simulink model "finalmodel1"  (R2024b)
settings: Solver=FixedStepDiscrete  StartTime=0.0  StopTime=110  FixedStep=SampleTime  MaxStep=1e-3  RelTol=1e-4  AbsTol=1e-3
InitFcn:
  | Ts=50e-6; SampleTime=50e-6; PSSMODEL=1;
  | MB=[1   0.2 30   1.25 40    12 160];
  | 
  | k=[8.3222    2.6014   19.0811    1.9818    3.6841   19.1783  240.6785    2.5684    4.3666   58.7391 7.6960   47.7975    8.7139  296.2463    2.7543    6.5051   47.7755    0.4780   35.4950   18.1866 94.2186]
  | k1=k(1);
  | k2=k(2);
  | k3=k(3);
  | k4=k(4);
  | k5=k(5);
  | k6=k(6);
  | k7=k(7);
  | k8=k(8);
  | k9=k(9);
  | k10=k(10);
  | k11=k(11);
  | k12=k(12);
  | k13=k(13);
  | k14=k(14);
  | k15=k(15);
  | k16=k(16);
  | k17=k(17);
  | k18=k(18);
  | k19=k(19);
  | k20=k(20);
  | k21=k(21);
undefined symbols (not defined in the file or in its folder): dEgdT, DiscIntNeverNeededParam, EgRef, gcbh, Rsh_array5pc, sigbuilder_block, sps_rtmsupport, Tref_K, VT_ref
libraries: spsThreePhaseVIMeasurementLib x14, spsLoadFlowBusLib x9, spsThreePhasePISectionLineLib x6, spsSeriesRLCBranchLib x5, spsThreePhaseTransformerTwoWindingsLib x4, slpidlib x4, spsThreePhaseParallelRLCLoadLib x4, spsThreePhaseSeriesRLCBranchLib x3, spsAlphaBetaZerotodq0Lib x2, spsSynchronousMachinepuStandardLib x2, spsExcitationSystemLib x2, spsMultiBandPowerSystemStabilizerLib x2
(part 9 of 9)

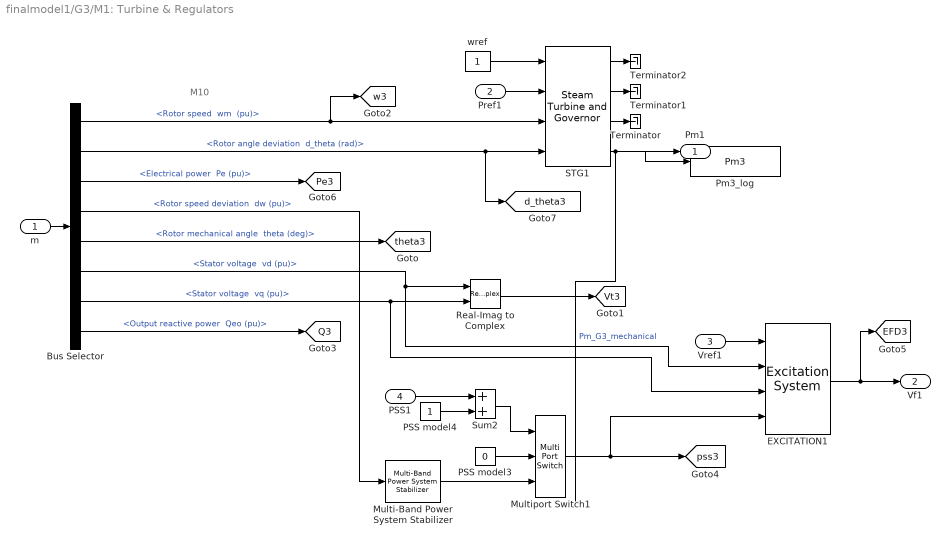
== system finalmodel1/G3/M1: Turbine & Regulators ==
  note: M10
  m : Inport  SampleTime=SampleTime
  Pref1 : Inport  Port=2  SampleTime=SampleTime
  Vref1 : Inport  Port=3  SampleTime=SampleTime
  PSS1 : Inport  Port=4  SampleTime=SampleTime
  Bus Selector : BusSelector  OutputSignals="Mechanical.Rotor speed  wm  (pu),Mechanical.Rotor angle deviation  d_theta (rad),Mechanical.Electrical power  Pe (pu),Mechanical.Rotor speed deviation  dw (pu),Mechanical.Rotor mechanical angle  theta (deg),dq0 components.Stator voltage  vd (pu),dq0 components.Stator voltage  vq (pu),Output reactive power  Qeo (pu)"
  EXCITATION1 : spsExcitationSystemLib/Excitation System  tr=0.01  reg=[20 .2]  exc=[ 1, 0.314 ]  tgr=[ 10 1]  damp=[ 0.063, 0.35 ]  sat=[ 0, 0 ]  lim="[ -5 5  0 ]"  v0=[1.025 1.2647]
      link override Model: Ts=SampleTime
      link override Model/Damping kfd.s // (tfd.s +1)/1st-Order Discrete Filter: Ts=SampleTime
      link override Model/Damping kfd.s // (tfd.s +1)/1st-Order Discrete Filter/Discrete State-Space: SampleTime=SampleTime
      link override Model/Exciter  1 // (te.s + ke)/1st order Lowpass: Ts=SampleTime
      link override Model/Exciter  1 // (te.s + ke)/1st order Lowpass/Discrete State-Space: SampleTime=SampleTime
      link override Model/Lead Lag Compensator tc.s+1 // tb.s+1: Ts=SampleTime
      link override Model/Lead Lag Compensator tc.s+1 // tb.s+1/Discrete State-Space: SampleTime=SampleTime
      link override Model/Low Pass Filter 1 // (tr.s +1) (with IC): Ts=SampleTime
      link override Model/Low Pass Filter 1 // (tr.s +1) (with IC)/Discrete State-Space: SampleTime=SampleTime
      link override Model/Main Regulator ka // (ta.s +1)/1st order Lowpass: Ts=SampleTime
      link override Model/Main Regulator ka // (ta.s +1)/1st order Lowpass/Discrete State-Space: SampleTime=SampleTime
      link override Model/Positive Sequence Voltage: Expr=sqrt(abs(u(1)^2 + u(2)^2))
      link override Model/Unit Delay1: SampleTime=SampleTime
      link override Model/Unit Delay2: SampleTime=SampleTime
      settings: LibrarySourceBlock=sps_lib/Electrical Machines/Synchronous Machine Control/Excitation System
  Multi-Band Power System Stabilizer : spsMultiBandPowerSystemStabilizerLib/Multi-Band Power System Stabilizer  OperationMode=Simplified settings  Kg=k1  GL=[k2 k3]  GI=[k4 k5]  GH=[k6 k7]  GLd=[66 66 9.4]  TcLF=[1.667 2 0 0 0 0 2 2.4 0 0 0 0 1 1]  GId=[66 66 47.6]  TcIF=[1 1 0.25 0.3 0 0 1 1 0.3 0.36 0 0 0 0]  GHd=[66 66 233]  TcHF="[0.01 0.012 0 0 0 0  0.012 0.0144 0 0 0 0 1 1]"  LIM=[.075 .15 .15 .15]  Plot_On=off  MagdB_On=off  FreqRange=logspace(-2,2,500)
      link override Model/Discrete Lead-Lag1: Ts=SampleTime
      link override Model/Discrete Lead-Lag1/Discrete State-Space: SampleTime=SampleTime
      link override Model/Discrete Lead-Lag2: Ts=SampleTime
      link override Model/Discrete Lead-Lag2/Discrete State-Space: SampleTime=SampleTime
      link override Model/Discrete Lead-Lag3: Ts=SampleTime
      link override Model/Discrete Lead-Lag3/Discrete State-Space: SampleTime=SampleTime
      link override Model/Discrete Lead-Lag4: Ts=SampleTime
      link override Model/Discrete Lead-Lag4/Discrete State-Space: SampleTime=SampleTime
      link override Model/Discrete Lead-Lag5: Ts=SampleTime
      link override Model/Discrete Lead-Lag5/Discrete State-Space: SampleTime=SampleTime
      link override Model/Discrete Lead-Lag6: Ts=SampleTime
      link override Model/Discrete Lead-Lag6/Discrete State-Space: SampleTime=SampleTime
      link override Model/HF speed sensor: Ts=SampleTime
      link override Model/HF speed sensor/Discrete State-Space: SampleTime=SampleTime
      link override Model/LF and IF speed sensor: Ts=SampleTime
      link override Model/LF and IF speed sensor/Discrete State-Space: SampleTime=SampleTime
      link override Model/Transfer function for detailed model (HF)/Transfer functions for detailed stabilizer/Discrete Lead-Lag1: Ts=SampleTime
      link override Model/Transfer function for detailed model (HF)/Transfer functions for detailed stabilizer/Discrete Lead-Lag1/Discrete State-Space: SampleTime=SampleTime
      link override Model/Transfer function for detailed model (HF)/Transfer functions for detailed stabilizer/Discrete Lead-Lag2: Ts=SampleTime
      link override Model/Transfer function for detailed model (HF)/Transfer functions for detailed stabilizer/Discrete Lead-Lag2/Discrete State-Space: SampleTime=SampleTime
      link override Model/Transfer function for detailed model (HF)/Transfer functions for detailed stabilizer1/Discrete Lead-Lag1: Ts=SampleTime
      link override Model/Transfer function for detailed model (HF)/Transfer functions for detailed stabilizer1/Discrete Lead-Lag1/Discrete State-Space: SampleTime=SampleTime
      link override Model/Transfer function for detailed model (HF)/Transfer functions for detailed stabilizer1/Discrete Lead-Lag2: Ts=SampleTime
      link override Model/Transfer function for detailed model (HF)/Transfer functions for detailed stabilizer1/Discrete Lead-Lag2/Discrete State-Space: SampleTime=SampleTime
      link override Model/Transfer function for detailed model (IF)/Transfer functions for detailed stabilizer/Discrete Lead-Lag1: Ts=SampleTime
      link override Model/Transfer function for detailed model (IF)/Transfer functions for detailed stabilizer/Discrete Lead-Lag1/Discrete State-Space: SampleTime=SampleTime
      link override Model/Transfer function for detailed model (IF)/Transfer functions for detailed stabilizer/Discrete Lead-Lag2: Ts=SampleTime
      link override Model/Transfer function for detailed model (IF)/Transfer functions for detailed stabilizer/Discrete Lead-Lag2/Discrete State-Space: SampleTime=SampleTime
      link override Model/Transfer function for detailed model (IF)/Transfer functions for detailed stabilizer1/Discrete Lead-Lag1: Ts=SampleTime
      link override Model/Transfer function for detailed model (IF)/Transfer functions for detailed stabilizer1/Discrete Lead-Lag1/Discrete State-Space: SampleTime=SampleTime
      link override Model/Transfer function for detailed model (IF)/Transfer functions for detailed stabilizer1/Discrete Lead-Lag2: Ts=SampleTime
      link override Model/Transfer function for detailed model (IF)/Transfer functions for detailed stabilizer1/Discrete Lead-Lag2/Discrete State-Space: SampleTime=SampleTime
      link override Model/Transfer function for detailed model (LF)/Transfer functions for detailed stabilizer/Discrete Lead-Lag1: Ts=SampleTime
      link override Model/Transfer function for detailed model (LF)/Transfer functions for detailed stabilizer/Discrete Lead-Lag1/Discrete State-Space: SampleTime=SampleTime
      link override Model/Transfer function for detailed model (LF)/Transfer functions for detailed stabilizer/Discrete Lead-Lag2: Ts=SampleTime
      link override Model/Transfer function for detailed model (LF)/Transfer functions for detailed stabilizer/Discrete Lead-Lag2/Discrete State-Space: SampleTime=SampleTime
      link override Model/Transfer function for detailed model (LF)/Transfer functions for detailed stabilizer1/Discrete Lead-Lag1: Ts=SampleTime
      link override Model/Transfer function for detailed model (LF)/Transfer functions for detailed stabilizer1/Discrete Lead-Lag1/Discrete State-Space: SampleTime=SampleTime
      link override Model/Transfer function for detailed model (LF)/Transfer functions for detailed stabilizer1/Discrete Lead-Lag2: Ts=SampleTime
      link override Model/Transfer function for detailed model (LF)/Transfer functions for detailed stabilizer1/Discrete Lead-Lag2/Discrete State-Space: SampleTime=SampleTime
      settings: LibrarySourceBlock=|
      | sps_lib/Electrical Machines/Synchronous Machine Control/Multi-Band
      | Power System Stabilizer
  Multiport Switch1 : MultiPortSwitch  Inputs=2  SampleTime=SampleTime  SaturateOnIntegerOverflow=off
  PSS model3 : Constant  Value=0  SampleTime=SampleTime
  PSS model4 : Constant  SampleTime=SampleTime
  Pm3_log : ToWorkspace  VariableName=Pm3  SaveFormat=Timeseries  SampleTime=-1
  Real-Imag to Complex : RealImagToComplex  SampleTime=SampleTime
  STG1 : spsSteamTurbineandGovernorLib/Steam Turbine and Governor  gentype=Tandem-compound (single mass)  reg1="[ 1  0.05    0 ]"  reg2="[ 0.001  0.15 ]"  reg3="[ -0.1  0.1  0  4.496 ]"  N=3600  turb1="[ 0  10   3.3   0.5   ]"  turb2="[   0   0.36    0.36   0.28   ]"  HA="[ 0.046  1.430  1.465   0.192 ]"  KA="[ 90.44  53.88  64.59   62.94  ]"  DA="[ 0.0115  0.3575  0.3663   0.0137  ]"  ini1=0.66512  ini2=[0.779316,-31.4247]
      link override Model/4 mass shaft/1 mass/Mass2: Ts=SampleTime
      link override Model/4 mass shaft/1 mass/Mass2/Ad*x(k-1): SampleTime=SampleTime
      link override Model/4 mass shaft/1 mass/Mass2/Bd*(u(k)+ u(k-1)): SampleTime=SampleTime
      link override Model/4 mass shaft/1 mass/Mass2/Delay_u: SampleTime=SampleTime
      link override Model/4 mass shaft/1 mass/Mass2/Delay_x: SampleTime=SampleTime
      link override Model/4 mass shaft/1 mass/Mass2/Digital Clock: SampleTime=SampleTime
      link override Model/4 mass shaft/1 mass/Mass2/Prediction/Unit Delay3: SampleTime=SampleTime
      link override Model/4 mass shaft/2 masses/Mass2: Ts=SampleTime
      link override Model/4 mass shaft/2 masses/Mass2/Ad*x(k-1): SampleTime=SampleTime
      link override Model/4 mass shaft/2 masses/Mass2/Bd*(u(k)+ u(k-1)): SampleTime=SampleTime
      link override Model/4 mass shaft/2 masses/Mass2/Delay_u: SampleTime=SampleTime
      link override Model/4 mass shaft/2 masses/Mass2/Delay_x: SampleTime=SampleTime
      link override Model/4 mass shaft/2 masses/Mass2/Digital Clock: SampleTime=SampleTime
      link override Model/4 mass shaft/2 masses/Mass2/Prediction/Unit Delay3: SampleTime=SampleTime
      link override Model/4 mass shaft/2 masses/Mass3: Ts=SampleTime
      link override Model/4 mass shaft/2 masses/Mass3/Ad*x(k-1): SampleTime=SampleTime
      link override Model/4 mass shaft/2 masses/Mass3/Bd*(u(k)+ u(k-1)): SampleTime=SampleTime
      link override Model/4 mass shaft/2 masses/Mass3/Delay_u: SampleTime=SampleTime
      link override Model/4 mass shaft/2 masses/Mass3/Delay_x: SampleTime=SampleTime
      link override Model/4 mass shaft/2 masses/Mass3/Digital Clock: SampleTime=SampleTime
      link override Model/4 mass shaft/2 masses/Mass3/Prediction/Unit Delay3: SampleTime=SampleTime
      link override Model/4 mass shaft/3 masses/Mass2: Ts=SampleTime
      link override Model/4 mass shaft/3 masses/Mass2/Ad*x(k-1): SampleTime=SampleTime
      link override Model/4 mass shaft/3 masses/Mass2/Bd*(u(k)+ u(k-1)): SampleTime=SampleTime
      link override Model/4 mass shaft/3 masses/Mass2/Delay_u: SampleTime=SampleTime
      link override Model/4 mass shaft/3 masses/Mass2/Delay_x: SampleTime=SampleTime
      link override Model/4 mass shaft/3 masses/Mass2/Digital Clock: SampleTime=SampleTime
      link override Model/4 mass shaft/3 masses/Mass2/Prediction/Unit Delay3: SampleTime=SampleTime
      link override Model/4 mass shaft/3 masses/Mass3: Ts=SampleTime
      link override Model/4 mass shaft/3 masses/Mass3/Ad*x(k-1): SampleTime=SampleTime
      link override Model/4 mass shaft/3 masses/Mass3/Bd*(u(k)+ u(k-1)): SampleTime=SampleTime
      link override Model/4 mass shaft/3 masses/Mass3/Delay_u: SampleTime=SampleTime
      link override Model/4 mass shaft/3 masses/Mass3/Delay_x: SampleTime=SampleTime
      link override Model/4 mass shaft/3 masses/Mass3/Digital Clock: SampleTime=SampleTime
      link override Model/4 mass shaft/3 masses/Mass3/Prediction/Unit Delay3: SampleTime=SampleTime
      link override Model/4 mass shaft/3 masses/Mass4: Ts=SampleTime
      link override Model/4 mass shaft/3 masses/Mass4/Ad*x(k-1): SampleTime=SampleTime
      link override Model/4 mass shaft/3 masses/Mass4/Bd*(u(k)+ u(k-1)): SampleTime=SampleTime
      link override Model/4 mass shaft/3 masses/Mass4/Delay_u: SampleTime=SampleTime
      link override Model/4 mass shaft/3 masses/Mass4/Delay_x: SampleTime=SampleTime
      link override Model/4 mass shaft/3 masses/Mass4/Digital Clock: SampleTime=SampleTime
      link override Model/4 mass shaft/3 masses/Mass4/Prediction/Unit Delay3: SampleTime=SampleTime
      link override Model/4 mass shaft/4 masses/Mass2: Ts=SampleTime
      link override Model/4 mass shaft/4 masses/Mass2/Ad*x(k-1): SampleTime=SampleTime
      link override Model/4 mass shaft/4 masses/Mass2/Bd*(u(k)+ u(k-1)): SampleTime=SampleTime
      link override Model/4 mass shaft/4 masses/Mass2/Delay_u: SampleTime=SampleTime
      link override Model/4 mass shaft/4 masses/Mass2/Delay_x: SampleTime=SampleTime
      link override Model/4 mass shaft/4 masses/Mass2/Digital Clock: SampleTime=SampleTime
      link override Model/4 mass shaft/4 masses/Mass2/Prediction/Unit Delay3: SampleTime=SampleTime
      link override Model/4 mass shaft/4 masses/Mass3: Ts=SampleTime
      link override Model/4 mass shaft/4 masses/Mass3/Ad*x(k-1): SampleTime=SampleTime
      link override Model/4 mass shaft/4 masses/Mass3/Bd*(u(k)+ u(k-1)): SampleTime=SampleTime
      link override Model/4 mass shaft/4 masses/Mass3/Delay_u: SampleTime=SampleTime
      link override Model/4 mass shaft/4 masses/Mass3/Delay_x: SampleTime=SampleTime
      link override Model/4 mass shaft/4 masses/Mass3/Digital Clock: SampleTime=SampleTime
      link override Model/4 mass shaft/4 masses/Mass3/Prediction/Unit Delay3: SampleTime=SampleTime
      link override Model/4 mass shaft/4 masses/Mass4: Ts=SampleTime
      link override Model/4 mass shaft/4 masses/Mass4/Ad*x(k-1): SampleTime=SampleTime
      link override Model/4 mass shaft/4 masses/Mass4/Bd*(u(k)+ u(k-1)): SampleTime=SampleTime
      link override Model/4 mass shaft/4 masses/Mass4/Delay_u: SampleTime=SampleTime
      link override Model/4 mass shaft/4 masses/Mass4/Delay_x: SampleTime=SampleTime
      link override Model/4 mass shaft/4 masses/Mass4/Digital Clock: SampleTime=SampleTime
      link override Model/4 mass shaft/4 masses/Mass4/Prediction/Unit Delay3: SampleTime=SampleTime
      link override Model/4 mass shaft/4 masses/Mass5: Ts=SampleTime
      link override Model/4 mass shaft/4 masses/Mass5/Ad*x(k-1): SampleTime=SampleTime
      link override Model/4 mass shaft/4 masses/Mass5/Bd*(u(k)+ u(k-1)): SampleTime=SampleTime
      link override Model/4 mass shaft/4 masses/Mass5/Delay_u: SampleTime=SampleTime
      link override Model/4 mass shaft/4 masses/Mass5/Delay_x: SampleTime=SampleTime
      link override Model/4 mass shaft/4 masses/Mass5/Digital Clock: SampleTime=SampleTime
      link override Model/4 mass shaft/4 masses/Mass5/Prediction/Unit Delay3: SampleTime=SampleTime
      link override Model/speed regulator/Servo-motor Position: SampleTime=SampleTime
      link override Model/speed regulator/Speed Relay: Ts=SampleTime
      link override Model/speed regulator/Speed Relay/In: SampleTime=SampleTime
      link override Model/speed regulator/Speed Relay/Model/Delay_x: SampleTime=SampleTime
      link override Model/speed regulator/Speed Relay/Out: SampleTime=SampleTime
      link override Model/steam turbine/Stage 1/Constant4: SampleTime=SampleTime
      link override Model/steam turbine/Stage 1/Stage1/Stage1: Ts=SampleTime
      link override Model/steam turbine/Stage 1/Stage1/Stage1/In: SampleTime=SampleTime
      link override Model/steam turbine/Stage 1/Stage1/Stage1/Model/Delay_x: SampleTime=SampleTime
      link override Model/steam turbine/Stage 1/Stage1/Stage1/Out: SampleTime=SampleTime
      link override Model/steam turbine/Stage 2 /Constant3: SampleTime=SampleTime
      link override Model/steam turbine/Stage 2 /Stage2/Stage2: Ts=SampleTime
      link override Model/steam turbine/Stage 2 /Stage2/Stage2/In: SampleTime=SampleTime
      link override Model/steam turbine/Stage 2 /Stage2/Stage2/Model/Delay_x: SampleTime=SampleTime
      link override Model/steam turbine/Stage 2 /Stage2/Stage2/Out: SampleTime=SampleTime
      link override Model/steam turbine/Stage 3/Constant2: SampleTime=SampleTime
      link override Model/steam turbine/Stage 3/Stage3/Stage3: Ts=SampleTime
      link override Model/steam turbine/Stage 3/Stage3/Stage3/In: SampleTime=SampleTime
      link override Model/steam turbine/Stage 3/Stage3/Stage3/Model/Delay_x: SampleTime=SampleTime
      link override Model/steam turbine/Stage 3/Stage3/Stage3/Out: SampleTime=SampleTime
      link override Model/steam turbine/Stage 4/Constant1: SampleTime=SampleTime
      link override Model/steam turbine/Stage 4/Stage4/Stage4: Ts=SampleTime
      link override Model/steam turbine/Stage 4/Stage4/Stage4/In: SampleTime=SampleTime
      link override Model/steam turbine/Stage 4/Stage4/Stage4/Model/Delay_x: SampleTime=SampleTime
      link override Model/steam turbine/Stage 4/Stage4/Stage4/Out: SampleTime=SampleTime
      settings: LibrarySourceBlock=|
      | sps_lib/Electrical Machines/Synchronous Machine Control/Steam Turbine
      | and Governor
  Sum2 : Sum  InputSameDT=on  SaturateOnIntegerOverflow=on  SampleTime=SampleTime  OutDataTypeStr=Inherit: Same as first input
  Terminator : Terminator
  Terminator1 : Terminator
  Terminator2 : Terminator
  wref : Constant  SampleTime=SampleTime
  Pm1 : Outport  SampleTime=SampleTime  InitialOutput=0
  Vf1 : Outport  Port=2  SampleTime=SampleTime  InitialOutput=0
  tag scope: EFD3=global, Pe3=global, Q3=global, Vt3=global, d_theta3=global, pss3=global, theta3=global, w3=global
  wires:
  Bus Selector/4 -> Multi-Band Power System Stabilizer/1  "<Rotor speed deviation  dw (pu)>"
  Multiport Switch1/1 -> EXCITATION1/4, [pss3]
  PSS model3/1 -> Multiport Switch1/2
  Multi-Band Power System Stabilizer/1 -> Multiport Switch1/3
  PSS model4/1 -> Sum2/2
  Sum2/1 -> Multiport Switch1/1
  PSS1/1 -> Sum2/1
  Bus Selector/8 -> [Q3]  "<Output reactive power  Qeo (pu)>"
  Bus Selector/3 -> [Pe3]  "<Electrical power  Pe (pu)>"
  Bus Selector/2 -> STG1/4, [d_theta3]  "<Rotor angle deviation  d_theta (rad)>"
  Bus Selector/1 -> STG1/3, [w3]  "<Rotor speed  wm  (pu)>"
  STG1/1 -> Terminator2/1
  STG1/2 -> Terminator1/1
  STG1/3 -> Terminator/1
  Bus Selector/6 -> EXCITATION1/2, Real-Imag to Complex/1  "<Stator voltage  vd (pu)>"
  Bus Selector/5 -> [theta3]  "<Rotor mechanical angle  theta (deg)>"
  Real-Imag to Complex/1 -> [Vt3]
  EXCITATION1/1 -> [EFD3], Vf1/1
  Vref1/1 -> EXCITATION1/1
  m/1 -> Bus Selector/1
  Pref1/1 -> STG1/2
  wref/1 -> STG1/1
  Bus Selector/7 -> Real-Imag to Complex/2, EXCITATION1/3  "<Stator voltage  vq (pu)>"
  STG1/4 -> Pm1/1, Pm3_log/1  "Pm_G3_mechanical"

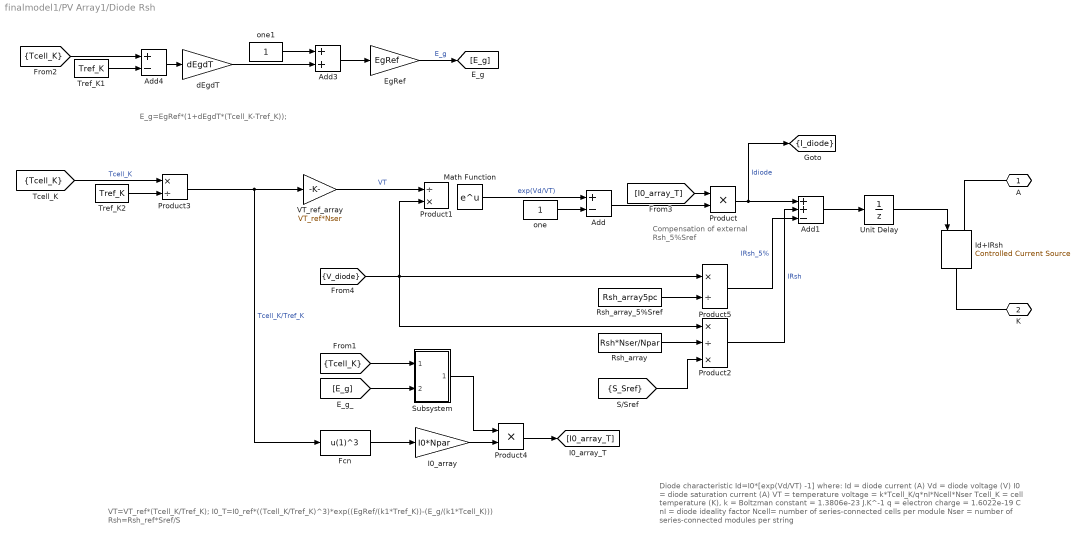
== system finalmodel1/PV Array1/Diode Rsh ==
  note: E_g=EgRef*(1+dEgdT*(Tcell_K-Tref_K));
  note: VT=VT_ref*(Tcell_K/Tref_K);
      | I0_T=I0_ref*((Tcell_K/Tref_K)^3)*exp((EgRef/(k1*Tref_K))-(E_g/(k1*Tcell_K)))
      | Rsh=Rsh_ref*Sref/S
  note: Diode characteristic
      |    Id=I0*[exp(Vd/VT) -1]
      |
      | where:
      |      Id = diode current (A)
      |      Vd = diode voltage (V)
      |      I0 = diode saturation current (A)
      |      VT = temperature voltage = k*Tcell_K/q*nI*Ncell*Nser
      | Tcell_K = cell temperature (K),
      |       k = Boltzman constant = 1.3806e-23 J.K^-1
      |       q = electron charge = 1.6022e-19 C
      |      nI = diode ideality factor
      |    Ncell= number of series-connected cells per module
      |    Nser = number of series-connected modules per string
  note: Compensation of
      | external Rsh_5%Sref
  Add : Sum  Inputs=+-
  Add1 : Sum  Inputs=++-
  Add3 : Sum
  Add4 : Sum  Inputs=+-
  EgRef : Gain  Gain=EgRef
  Fcn : Fcn  Expr=u(1)^3
  I0_array : Gain  Gain=I0*Npar
  Id+IRsh : spsControlledCurrentSourceLib/Controlled Current Source  Initialize=on  Source_Type=AC  Amplitude=0  Phase=0  Frequency=0  Measurements=None
  Math Function : Math  SignedPower=on  OutputSignalType=real
  Product : Product  RndMeth=Zero
  Product1 : Product  Inputs=/*  RndMeth=Zero
  Product2 : Product  Inputs=*/*  RndMeth=Zero
  Product3 : Product  Inputs=*/  RndMeth=Zero
  Product4 : Product  Inputs=**  RndMeth=Zero
  Product5 : Product  Inputs=*/  RndMeth=Zero
  Rsh_array : Constant  Value=Rsh*Nser/Npar
  Rsh_array_5%Sref : Constant  Value=Rsh_array5pc
  Subsystem : Subsystem
  Tref_K1 : Constant  Value=Tref_K
  Tref_K2 : Constant  Value=Tref_K
  Unit Delay : UnitDelay  SampleTime=SampleTime  HasFrameUpgradeWarning=on
  VT_ref_array : Gain  Gain=VT_ref*Nser
  dEgdT : Gain  Gain=dEgdT
  one : Constant
  one1 : Constant
  A : PMIOPort  Side=Left
  K : PMIOPort  Port=2  Side=Right
  tag scope: I_diode=scoped
  wires:
  [V_diode] -> Product2/1, Product5/1, Product1/2
  [S_Sref] -> Product2/3
  [I0_array_T] -> Product/1
  VT_ref_array/1 -> Product1/1  "VT"
  Add/1 -> Product/2
  Product4/1 -> [I0_array_T]
  Tref_K2/1 -> Product3/2
  [E_g] -> Subsystem/2(E_g)
  [Tcell_K] -> Subsystem/1(Tcell_K)
  Subsystem/1(exp) -> Product4/1
  Tref_K1/1 -> Add4/2
  [Tcell_K] -> Add4/1
  Fcn/1 -> I0_array/1
  I0_array/1 -> Product4/2
  EgRef/1 -> [E_g]  "E_g"
  Add3/1 -> EgRef/1
  dEgdT/1 -> Add3/2
  Add4/1 -> dEgdT/1
  one1/1 -> Add3/1
  Product3/1 -> Fcn/1, VT_ref_array/1  "Tcell_K/Tref_K"
  [Tcell_K] -> Product3/1  "Tcell_K"
  Rsh_array/1 -> Product2/2
  one/1 -> Add/2
  Product/1 -> [I_diode], Add1/1  "Idiode"
  Product2/1 -> Add1/2  "IRsh"
  Math Function/1 -> Add/1  "exp(Vd/VT)"
  Rsh_array_5%Sref/1 -> Product5/2
  Product5/1 -> Add1/3  "IRsh_5%"
  Add1/1 -> Unit Delay/1
  Unit Delay/1 -> Id+IRsh/1
  connections:
  A/RConn1 -- Id+IRsh/LConn1
  Id+IRsh/RConn1 -- K/RConn1

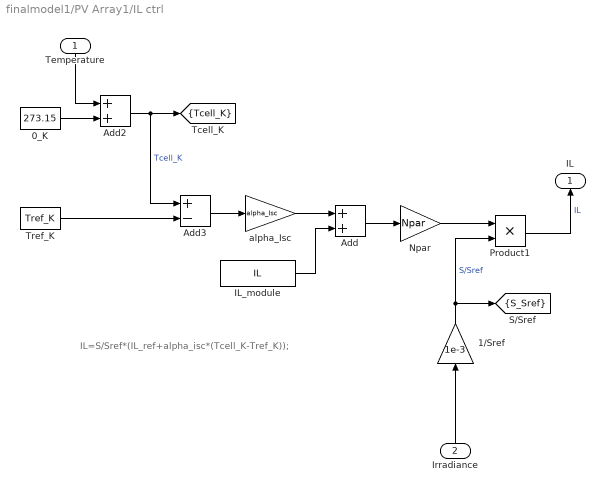
== system finalmodel1/PV Array1/IL ctrl ==
  note: IL=S/Sref*(IL_ref+alpha_isc*(Tcell_K-Tref_K));
  Temperature : Inport
  Irradiance : Inport  Port=2
  0_K : Constant  Value=273.15
  1/Sref : Gain  Gain=1e-3
  Add : Sum
  Add2 : Sum
  Add3 : Sum  Inputs=+-
  IL_module : Constant  Value=IL
  Npar : Gain  Gain=Npar
  Product1 : Product  Inputs=**  RndMeth=Zero
  Tref_K : Constant  Value=Tref_K
  alpha_Isc : Gain  Gain=alpha_Isc
  IL : Outport  VectorParamsAs1DForOutWhenUnconnected=off
  tag scope: S_Sref=scoped, Tcell_K=scoped
  wires:
  1/Sref/1 -> [S_Sref], Product1/2  "S/Sref"
  Npar/1 -> Product1/1
  Add2/1 -> [Tcell_K], Add3/1  "Tcell_K"
  Add/1 -> Npar/1
  0_K/1 -> Add2/2
  IL_module/1 -> Add/2
  Product1/1 -> IL/1  "IL"
  Tref_K/1 -> Add3/2
  Add3/1 -> alpha_Isc/1
  alpha_Isc/1 -> Add/1
  Irradiance/1 -> 1/Sref/1
  Temperature/1 -> Add2/1

== system finalmodel1/PV Array1/Vdiode ==
  note: Vd=V_PV + Rs*I_PV
  I_PV : Inport
  V_PV : Inport  Port=2
  Add1 : Sum
  Product2 : Product  Inputs=**  RndMeth=Zero
  Rs_array_ : Constant  Value=Rs*Nser/Npar
  Vd : Outport  VectorParamsAs1DForOutWhenUnconnected=off
  wires:
  Add1/1 -> Vd/1  "Vd"
  I_PV/1 -> Product2/1
  Product2/1 -> Add1/2
  V_PV/1 -> Add1/1
  Rs_array_/1 -> Product2/2

== system finalmodel1/PV Array1/Diode Rsh/Subsystem ==
  note: exp((EgRef/(k1*Tref_K))-(E_g/(k1*Tcell_K)))
  Tcell_K : Inport
  E_g : Inport  Port=2
  Add : Sum  Inputs=+-
  EgRef : Constant  Value=EgRef/(k1*Tref_K)
  Math Function : Math  SignedPower=on  OutputSignalType=real
  Product : Product  Inputs=*/
  k1 : Gain  Gain=k1
  exp : Outport  VectorParamsAs1DForOutWhenUnconnected=off
  wires:
  Math Function/1 -> exp/1
  Product/1 -> Add/2
  k1/1 -> Product/2
  Tcell_K/1 -> k1/1
  E_g/1 -> Product/1
  EgRef/1 -> Add/1

== matlab function finalmodel1/P&O ==
  settings: updateMethod=DISCRETE  sampleTime=1e-4
  data: Vpv input; D output; Ipv input
function D = PO(Vpv,Ipv)
 Dmax=0.9;
 Dmin=0.1;
 Dinit=0.9;
 deltaD=1e-3;
 persistent Dpre Ppre Vpre;
 
 %first run
     if isempty(Dpre)
         Dpre=Dinit;
         Vpre=0;
         Ppre=0;
     end
 Ppv=Vpv*Ipv;
 dp=Ppv-Ppre;
 dv=Vpv-Vpre;
 
     if dp~=0 
             if(dp>0)
                     if(dv<0)
                         D=Dpre+deltaD;
                     else
                         D=Dpre-deltaD;
                     end     
             else                   
                     if(dv<0)
                         D=Dpre-deltaD;
                     else
                         D=Dpre+deltaD;
                     end
             end   
    else
          D=Dpre;
    end
    
    if D>=Dmax || D <= Dmin
        D=Dpre;
    end
    
    Ppre=Ppv;
    Vpre=Vpv;
    Dpre=D;
end
